simulink model "SafeBeat_v1_step11_test"  (R2019a)
settings: Solver=FixedStepDiscrete  StartTime=0.0  StopTime=10.0  FixedStep=0.027778  RelTol=1e-3
libraries: simulink x6, dsparch4 x1
settings Model: Creator=Admin  LastModifiedBy=Admin

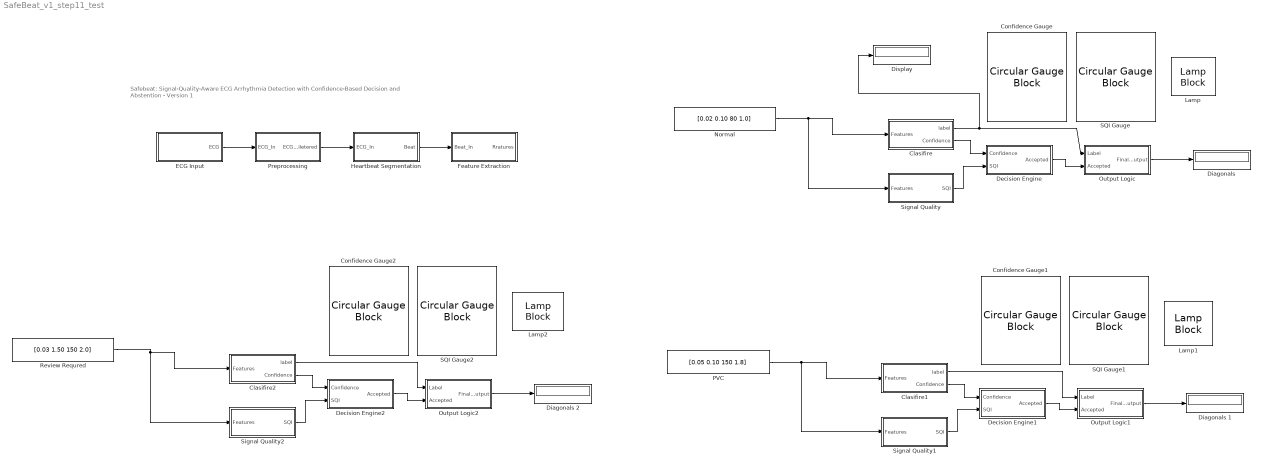
== system SafeBeat_v1_step11_test ==
  note: Safebeat: Signal-Quality-Aware ECG Arrhythmia Detection with Confidence-Based Decision and Abstention - Version 1
  Clasifire : Subsystem
  Clasifire1 : Subsystem
  Clasifire2 : Subsystem
  Confidence Gauge : CircularGaugeBlock  ScaleMax=1
  Confidence Gauge1 : CircularGaugeBlock  ScaleMax=1
  Confidence Gauge2 : CircularGaugeBlock  ScaleMax=1
  Decision Engine : Subsystem
  Decision Engine1 : Subsystem
  Decision Engine2 : Subsystem
  "Diagonals " : Display
  Diagonals 1 : Display
  Diagonals 2 : Display
  Display : Display
  ECG Input : Subsystem
  Feature Extraction : Subsystem
  Heartbeat Segmentation : Subsystem
  Lamp : LampBlock
  Lamp1 : LampBlock
  Lamp2 : LampBlock  LabelPosition=Bottom
  Normal : Constant  Value=[0.02 0.10 80 1.0]
  Output Logic : Subsystem
  Output Logic1 : Subsystem
  Output Logic2 : Subsystem
  PVC : Constant  Value=[0.05 0.10 150 1.8]
  Preprocessing : Subsystem
  Review Requred : Constant  Value=[0.03 1.50 150 2.0]
  SQI Gauge : CircularGaugeBlock  ScaleMax=1
  SQI Gauge1 : CircularGaugeBlock  ScaleMax=1
  SQI Gauge2 : CircularGaugeBlock  ScaleMax=1
  Signal Quality : Subsystem
  Signal Quality1 : Subsystem
  Signal Quality2 : Subsystem
  wires:
  ECG Input/1(ECG) -> Preprocessing/1(ECG_In)
  Preprocessing/1(ECG_Filetered) -> Heartbeat Segmentation/1(ECG_In)
  Heartbeat Segmentation/1("Beat ") -> Feature Extraction/1(Beat_In)
  Signal Quality/1(SQI) -> Decision Engine/2(SQI)
  Decision Engine/1(Accepted) -> Output Logic/2(Accepted)
  Output Logic/1(FinalOutput) -> "Diagonals "/1
  Normal/1 -> Signal Quality/1(Features), Clasifire/1(Features)
  Signal Quality1/1(SQI) -> Decision Engine1/2(SQI)
  PVC/1 -> Clasifire1/1(Features), Signal Quality1/1(Features)
  Decision Engine1/1(Accepted) -> Output Logic1/2(Accepted)
  Output Logic1/1(FinalOutput) -> Diagonals 1/1
  Clasifire/1(label) -> Display/1, Output Logic/1(Label)
  Clasifire/2(Confidence) -> Decision Engine/1(Confidence)
  Clasifire1/1(label) -> Output Logic1/1(Label)
  Clasifire1/2(Confidence) -> Decision Engine1/1(Confidence)
  Clasifire2/1(label) -> Output Logic2/1(Label)
  Output Logic2/1(FinalOutput) -> Diagonals 2/1
  Clasifire2/2(Confidence) -> Decision Engine2/1(Confidence)
  Decision Engine2/1(Accepted) -> Output Logic2/2(Accepted)
  Review Requred/1 -> Clasifire2/1(Features), Signal Quality2/1(Features)
  Signal Quality2/1(SQI) -> Decision Engine2/2(SQI)

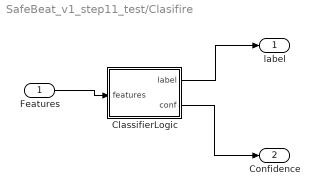
== system SafeBeat_v1_step11_test/Clasifire ==
  Features : Inport
  ClassifierLogic : MATLAB Function  TreatAsAtomicUnit=on
  label : Outport
  Confidence : Outport  Port=2
  wires:
  ClassifierLogic/1(label) -> label/1
  Features/1 -> ClassifierLogic/1(features)
  ClassifierLogic/2(conf) -> Confidence/1

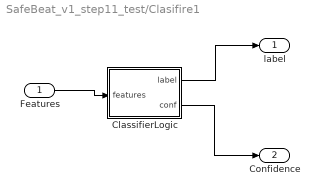
== system SafeBeat_v1_step11_test/Clasifire1 ==
  Features : Inport
  ClassifierLogic : MATLAB Function  TreatAsAtomicUnit=on
  label : Outport
  Confidence : Outport  Port=2
  wires:
  ClassifierLogic/1(label) -> label/1
  Features/1 -> ClassifierLogic/1(features)
  ClassifierLogic/2(conf) -> Confidence/1

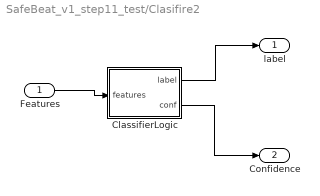
== system SafeBeat_v1_step11_test/Clasifire2 ==
  Features : Inport
  ClassifierLogic : MATLAB Function  TreatAsAtomicUnit=on
  label : Outport
  Confidence : Outport  Port=2
  wires:
  ClassifierLogic/1(label) -> label/1
  Features/1 -> ClassifierLogic/1(features)
  ClassifierLogic/2(conf) -> Confidence/1

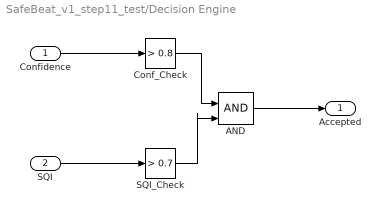
== system SafeBeat_v1_step11_test/Decision Engine ==
  Confidence : Inport
  SQI : Inport  Port=2
  AND : Logic  IconShape=distinctive  AllPortsSameDT=off  OutDataTypeStr=boolean
  Conf_Check : simulink/Logic and Bit Operations/Compare To Constant  relop=>  const=0.8  OutDataTypeStr=boolean
  SQI_Check : simulink/Logic and Bit Operations/Compare To Constant  relop=>  const=0.7  OutDataTypeStr=boolean
  Accepted : Outport
  wires:
  Confidence/1 -> Conf_Check/1
  Conf_Check/1 -> AND/1
  SQI/1 -> SQI_Check/1
  SQI_Check/1 -> AND/2
  AND/1 -> Accepted/1

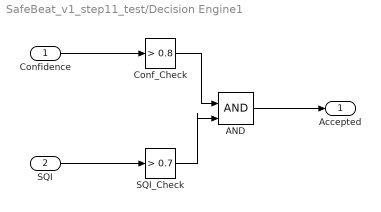
== system SafeBeat_v1_step11_test/Decision Engine1 ==
  Confidence : Inport
  SQI : Inport  Port=2
  AND : Logic  IconShape=distinctive  AllPortsSameDT=off  OutDataTypeStr=boolean
  Conf_Check : simulink/Logic and Bit Operations/Compare To Constant  relop=>  const=0.8  OutDataTypeStr=boolean
  SQI_Check : simulink/Logic and Bit Operations/Compare To Constant  relop=>  const=0.7  OutDataTypeStr=boolean
  Accepted : Outport
  wires:
  Confidence/1 -> Conf_Check/1
  Conf_Check/1 -> AND/1
  SQI/1 -> SQI_Check/1
  SQI_Check/1 -> AND/2
  AND/1 -> Accepted/1

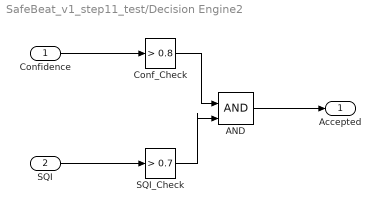
== system SafeBeat_v1_step11_test/Decision Engine2 ==
  Confidence : Inport
  SQI : Inport  Port=2
  AND : Logic  IconShape=distinctive  AllPortsSameDT=off  OutDataTypeStr=boolean
  Conf_Check : simulink/Logic and Bit Operations/Compare To Constant  relop=>  const=0.8  OutDataTypeStr=boolean
  SQI_Check : simulink/Logic and Bit Operations/Compare To Constant  relop=>  const=0.7  OutDataTypeStr=boolean
  Accepted : Outport
  wires:
  Confidence/1 -> Conf_Check/1
  Conf_Check/1 -> AND/1
  SQI/1 -> SQI_Check/1
  SQI_Check/1 -> AND/2
  AND/1 -> Accepted/1

== system SafeBeat_v1_step11_test/ECG Input ==
  "From Workspace " : FromWorkspace  VariableName=ecgSignal  SampleTime=0
  ECG : Outport
  wires:
  "From Workspace "/1 -> ECG/1

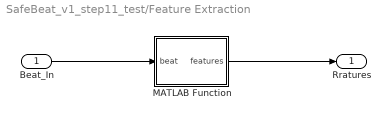
== system SafeBeat_v1_step11_test/Feature Extraction ==
  Beat_In : Inport
  MATLAB Function : MATLAB Function  TreatAsAtomicUnit=on
  Rratures : Outport
  wires:
  MATLAB Function/1(features) -> Rratures/1
  Beat_In/1 -> MATLAB Function/1(beat)

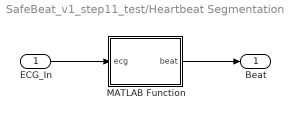
== system SafeBeat_v1_step11_test/Heartbeat Segmentation ==
  ECG_In : Inport
  MATLAB Function : MATLAB Function  TreatAsAtomicUnit=on
  "Beat " : Outport
  wires:
  ECG_In/1 -> MATLAB Function/1(ecg)
  MATLAB Function/1(beat) -> "Beat "/1

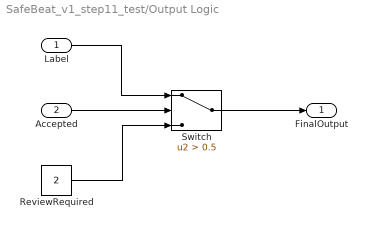
== system SafeBeat_v1_step11_test/Output Logic ==
  Label : Inport
  Accepted : Inport  Port=2
  ReviewRequired : Constant  Value=2
  Switch : Switch  Criteria=u2 > Threshold  Threshold=0.5
  FinalOutput : Outport
  wires:
  Switch/1 -> FinalOutput/1
  Label/1 -> Switch/1
  Accepted/1 -> Switch/2
  ReviewRequired/1 -> Switch/3

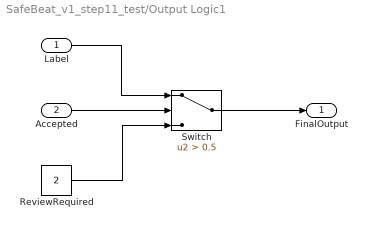
== system SafeBeat_v1_step11_test/Output Logic1 ==
  Label : Inport
  Accepted : Inport  Port=2
  ReviewRequired : Constant  Value=2
  Switch : Switch  Criteria=u2 > Threshold  Threshold=0.5
  FinalOutput : Outport
  wires:
  Switch/1 -> FinalOutput/1
  Label/1 -> Switch/1
  Accepted/1 -> Switch/2
  ReviewRequired/1 -> Switch/3

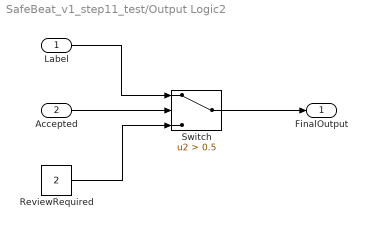
== system SafeBeat_v1_step11_test/Output Logic2 ==
  Label : Inport
  Accepted : Inport  Port=2
  ReviewRequired : Constant  Value=2
  Switch : Switch  Criteria=u2 > Threshold  Threshold=0.5
  FinalOutput : Outport
  wires:
  Switch/1 -> FinalOutput/1
  Label/1 -> Switch/1
  Accepted/1 -> Switch/2
  ReviewRequired/1 -> Switch/3

== system SafeBeat_v1_step11_test/Preprocessing ==
  ECG_In : Inport
  Digital Filter Design : dsparch4/Digital Filter Design  mwdsp_browser_bugfix_var=off
  ECG_Filetered : Outport
  wires:
  ECG_In/1 -> Digital Filter Design/1
  Digital Filter Design/1 -> ECG_Filetered/1

== system SafeBeat_v1_step11_test/Signal Quality ==
  Features : Inport
  SQICalculation : MATLAB Function  TreatAsAtomicUnit=on
  SQI : Outport
  wires:
  Features/1 -> SQICalculation/1(features)
  SQICalculation/1(sqi) -> SQI/1

== system SafeBeat_v1_step11_test/Signal Quality1 ==
  Features : Inport
  SQICalculation : MATLAB Function  TreatAsAtomicUnit=on
  SQI : Outport
  wires:
  Features/1 -> SQICalculation/1(features)
  SQICalculation/1(sqi) -> SQI/1

== system SafeBeat_v1_step11_test/Signal Quality2 ==
  Features : Inport
  SQICalculation : MATLAB Function  TreatAsAtomicUnit=on
  SQI : Outport
  wires:
  Features/1 -> SQICalculation/1(features)
  SQICalculation/1(sqi) -> SQI/1

== matlab function SafeBeat_v1_step11_test/Feature Extraction/MATLAB Function ==
  data: beat input; features output size=[4 1]
function features = fcn(beat)

meanVal = mean(beat);

stdVal = std(beat);

energyVal = sum(beat.^2);

peakVal = max(abs(beat));

features = [
    meanVal;
    stdVal;
    energyVal;
    peakVal
];

end

== matlab function SafeBeat_v1_step11_test/Heartbeat Segmentation/MATLAB Function ==
  data: ecg input; beat output size=[250 1]
function beat = fcn(ecg)

persistent buffer

if isempty(buffer)
    buffer = zeros(250,1);
end

buffer = [buffer(2:end); ecg];

beat = buffer;

== matlab function SafeBeat_v1_step11_test/Clasifire/ClassifierLogic ==
  data: features input; label output double size=1; conf output double size=1
function [label, conf] = classify(features)

energy = features(3);

if energy > 100

    label = 1;
    conf = 0.90;

else

    label = 0;
    conf = 0.85;

end

end

== matlab function SafeBeat_v1_step11_test/Signal Quality/SQICalculation ==
  data: features input; sqi output double size=1
function sqi = calcSQI(features)

noiseMetric = features(2);

sqi = 1/(1 + noiseMetric);

end

== matlab function SafeBeat_v1_step11_test/Clasifire1/ClassifierLogic ==
  data: features input; label output double size=1; conf output double size=1
function [label, conf] = classify(features)

energy = features(3);

if energy > 100

    label = 1;
    conf = 0.90;

else

    label = 0;
    conf = 0.85;

end

end

== matlab function SafeBeat_v1_step11_test/Signal Quality1/SQICalculation ==
  data: features input; sqi output double size=1
function sqi = calcSQI(features)

noiseMetric = features(2);

sqi = 1/(1 + noiseMetric);

end

== matlab function SafeBeat_v1_step11_test/Clasifire2/ClassifierLogic ==
  data: features input; label output double size=1; conf output double size=1
function [label, conf] = classify(features)

energy = features(3);

if energy > 100

    label = 1;
    conf = 0.90;

else

    label = 0;
    conf = 0.85;

end

end

== matlab function SafeBeat_v1_step11_test/Signal Quality2/SQICalculation ==
  data: features input; sqi output double size=1
function sqi = calcSQI(features)

noiseMetric = features(2);

sqi = 1/(1 + noiseMetric);

end
